simulink model "NREL5MW_FBSWE_SLOW2DOF_AdvancedTorqueController_Part1"  (R2021b)
settings: Solver=ode4  StartTime=0.0  StopTime=Parameter.Time.TMax  FixedStep=Parameter.Time.dt  RelTol=1e-3  EnableMultiTasking=on
values from neighbouring files (symbols this model uses):
  Parameter = NREL5MWDefaultParameter_FBSWE_AvancedTorqueController(Parameter)    [Exercise06_AdvancedTorqueControllerTest.m]    (also in Exercise06_AdvancedTorqueControllerTest_Part1.m = NREL5MWDefaultParameter_FBSWE_AvancedTorqueController_Part1(; Exercise06_SetPointFadingFineTuning.m = NREL5MWDefaultParameter_FBSWE_SetPointFading(Parameter); Exercise06_SetPointFadingFineTuning_Part3.m = NREL5MWDefaultParameter_FBSWE_SetPointFading_Part2(Parameter; Exercise06_SetPointFadingTest.m = NREL5MWDefaultParameter_FBSWE_SetPointFading(Parameter))
libraries: simulink x1
settings Model: Creator=Phoenix_Shao  LastModifiedBy=david
settings SolverCC: AlgebraicLoopSolver=TrustRegion
settings DataIOCC: MaxDataPoints=1000000  SaveFormat=Array  DSMLogging=off  ReturnWorkspaceOutputs=off
settings OptimizationCC: ExpressionDepthLimit=2147483647  InitFltsAndDblsToZero=on  EfficientMapNaN2IntZero=off  LifeSpan=inf
settings DebuggingCC: SaveWithParameterizedLinksMsg=none  UnderspecifiedInitializationDetection=Classic  MergeDetectMultiDrivingBlocksExec=none  SignalResolutionControl=TryResolveAllWithWarning  SolverPrmCheckMsg=warning  MultiTaskDSMMsg=warning  MultiTaskCondExecSysMsg=none  FcnCallInpInsideContextMsg=warning  AllowSymbolicDim=off  StateNameClashWarn=warning  SFUnexpectedBacktrackingDiag=warning  SFNoUnconditionalDefaultTransitionDiag=warning  SFExecutionAtInitializationDiag=none  SFMachineParentedDataDiag=warning  ArithmeticOperatorsInVariantConditions=warning
settings HardwareCC: ProdBitPerPointer=32  ProdBitPerSizeT=32  ProdBitPerPtrDiffT=32  ProdLargestAtomicFloat=None  ProdIntDivRoundTo=Undefined  ProdEndianess=Unspecified  ProdWordSize=32  ProdHWDeviceType=32-bit Generic  TargetBitPerPointer=64  TargetBitPerSizeT=64  TargetBitPerPtrDiffT=64  TargetLongLongMode=on  TargetIntDivRoundTo=Zero  TargetEndianess=LittleEndian  TargetWordSize=64  TargetHWDeviceType=MATLAB Host  ProdEqTarget=off
settings ModelReferenceCC: PropagateSignalLabelsOutOfModel=off
settings SFSimCC: SimUseLocalCustomCode=off  SimParseCustomCode=off  CustomCodeUndefinedFunction=UseInterfaceOnly
settings RTWCC: SystemTargetFile=accel.tlc  TemplateMakefile=accel_default_tmf  RTWVerbose=off  RTWUseLocalCustomCode=off
settings CodeAppCC: MaxIdLength=128  StateflowObjectComments=on
settings STFCustomTargetCC: MATLABClassNameForMDSCustomization=Simulink.SoftwareTarget.TargetSpecificTriggerConfigurationBase  SystemTargetFile=accel.tlc
settings ConfigComp: CovMetricSettings=dw  CovSaveCumulativeToWorkspaceVar=on  CovSaveSingleToWorkspaceVar=on  CovExternalEMLEnable=off

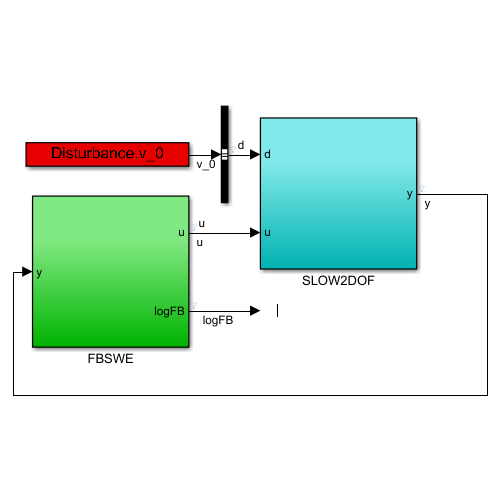
[thumbnail: Simulink's stored preview of the top-level diagram]
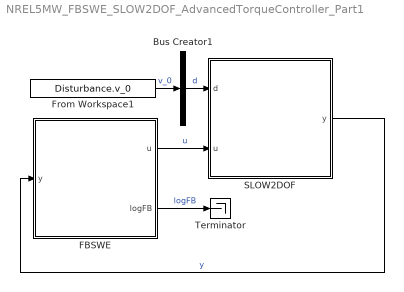
== system NREL5MW_FBSWE_SLOW2DOF_AdvancedTorqueController_Part1 ==
  Bus Creator1 : BusCreator  Inputs=1
  FBSWE : Subsystem
  From Workspace1 : FromWorkspace  VariableName=Disturbance.v_0
  SLOW2DOF : Subsystem
  Terminator : Terminator
  wires:
  FBSWE/1(u) -> SLOW2DOF/2(u)  "u"
  Bus Creator1/1 -> SLOW2DOF/1(d)  "d"
  From Workspace1/1 -> Bus Creator1/1  "v_0"
  SLOW2DOF/1(y) -> FBSWE/1(y)  "y"
  FBSWE/2(logFB) -> Terminator/1  "logFB"

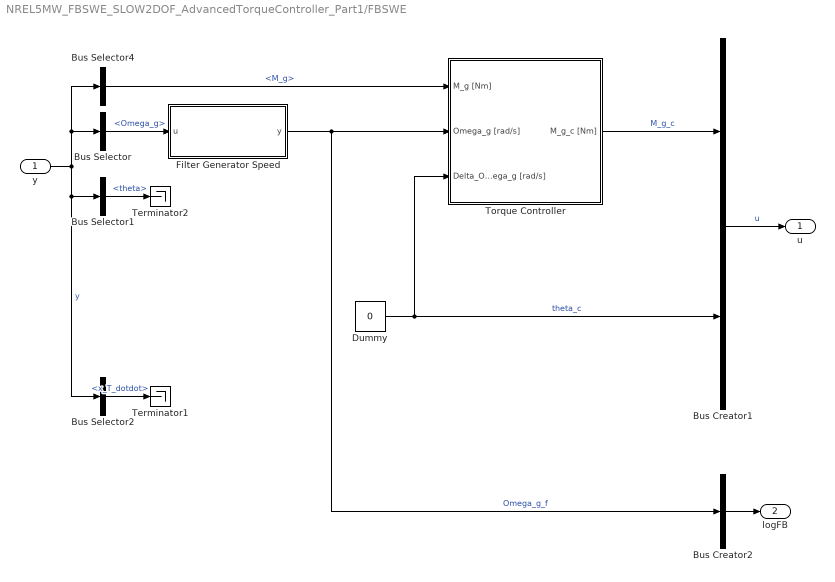
== system NREL5MW_FBSWE_SLOW2DOF_AdvancedTorqueController_Part1/FBSWE ==
  y : Inport
  Bus Creator1 : BusCreator  Inputs=2
  Bus Creator2 : BusCreator  Inputs=1
  Bus Selector : BusSelector  OutputSignals=Omega_g
  Bus Selector1 : BusSelector  OutputSignals=theta
  Bus Selector2 : BusSelector  OutputSignals=x_T_dotdot
  Bus Selector4 : BusSelector  OutputSignals=M_g
  Dummy : Constant  Value=0
  Filter Generator Speed : Subsystem
  Terminator1 : Terminator
  Terminator2 : Terminator
  Torque Controller : Subsystem
  u : Outport  VectorParamsAs1DForOutWhenUnconnected=off
  logFB : Outport  Port=2  VectorParamsAs1DForOutWhenUnconnected=off
  wires:
  Bus Selector/1 -> Filter Generator Speed/1(u)  "<Omega_g>"
  y/1 -> Bus Selector4/1, Bus Selector/1, Bus Selector2/1, Bus Selector1/1  "y"
  Torque Controller/1(M_g_c [Nm]) -> Bus Creator1/1  "M_g_c"
  Bus Creator1/1 -> u/1  "u"
  Filter Generator Speed/1(y) -> Torque Controller/2(Omega_g [rad/s]), Bus Creator2/1  "Omega_g_f"
  Bus Creator2/1 -> logFB/1
  Dummy/1 -> Torque Controller/3(Delta_Omega_g [rad/s]), Bus Creator1/2  "theta_c"
  Bus Selector2/1 -> Terminator1/1  "<x_T_dotdot>"
  Bus Selector1/1 -> Terminator2/1  "<theta>"
  Bus Selector4/1 -> Torque Controller/1(M_g [Nm])  "<M_g>"

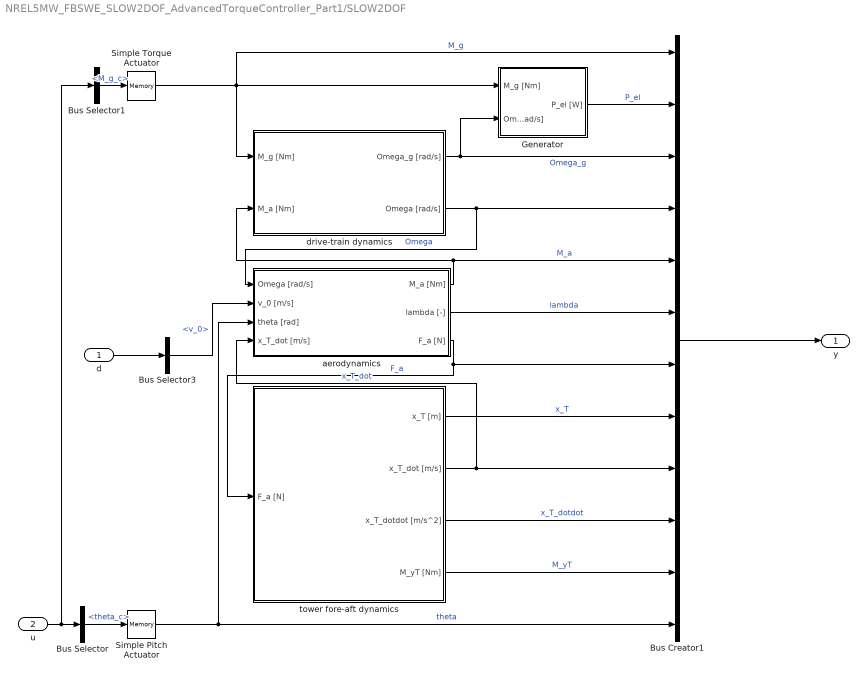
== system NREL5MW_FBSWE_SLOW2DOF_AdvancedTorqueController_Part1/SLOW2DOF ==
  d : Inport
  u : Inport  Port=2
  Bus Creator1 : BusCreator  Inputs=12
  Bus Selector : BusSelector  OutputSignals=theta_c
  Bus Selector1 : BusSelector  OutputSignals=M_g_c
  Bus Selector3 : BusSelector  OutputSignals=v_0
  Generator : Subsystem
  Simple Pitch Actuator : Memory  InitialCondition=Parameter.IC.theta
  Simple Torque Actuator : Memory  InitialCondition=Parameter.IC.M_g
  aerodynamics : Subsystem
  drive-train dynamics : Subsystem
  tower fore-aft dynamics : Subsystem
  y : Outport  VectorParamsAs1DForOutWhenUnconnected=off
  wires:
  Generator/1(P_el [W]) -> Bus Creator1/2  "P_el"
  Bus Creator1/1 -> y/1
  u/1 -> Bus Selector/1, Bus Selector1/1
  Bus Selector/1 -> Simple Pitch Actuator/1  "<theta_c>"
  aerodynamics/3(F_a [N]) -> Bus Creator1/7, tower fore-aft dynamics/1(F_a [N])  "F_a"
  aerodynamics/1(M_a [Nm]) -> Bus Creator1/5, drive-train dynamics/2(M_a [Nm])  "M_a"
  tower fore-aft dynamics/2(x_T_dot [m/s]) -> Bus Creator1/9, aerodynamics/4(x_T_dot [m/s])  "x_T_dot"
  drive-train dynamics/2(Omega [rad/s]) -> Bus Creator1/4, aerodynamics/1(Omega [rad/s])  "Omega"
  drive-train dynamics/1(Omega_g [rad/s]) -> Bus Creator1/3, Generator/2(Omega_g [rad/s])  "Omega_g"
  d/1 -> Bus Selector3/1
  Bus Selector3/1 -> aerodynamics/2(v_0 [m/s])  "<v_0>"
  Simple Pitch Actuator/1 -> Bus Creator1/12, aerodynamics/3(theta [rad])  "theta"
  Bus Selector1/1 -> Simple Torque Actuator/1  "<M_g_c>"
  aerodynamics/2(lambda [-]) -> Bus Creator1/6  "lambda"
  tower fore-aft dynamics/1(x_T [m]) -> Bus Creator1/8  "x_T"
  tower fore-aft dynamics/3(x_T_dotdot [m/s^2]) -> Bus Creator1/10  "x_T_dotdot"
  tower fore-aft dynamics/4(M_yT [Nm]) -> Bus Creator1/11  "M_yT"
  Simple Torque Actuator/1 -> Bus Creator1/1, Generator/1(M_g [Nm]), drive-train dynamics/1(M_g [Nm])  "M_g"

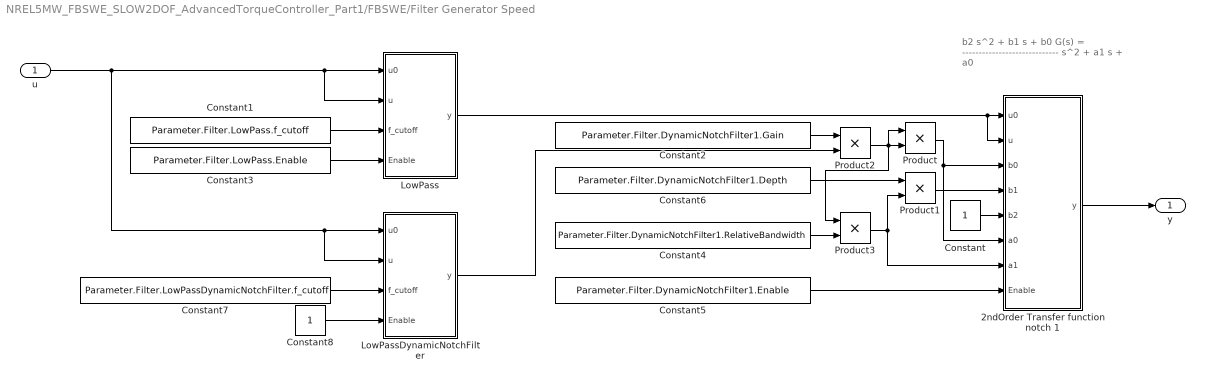
== system NREL5MW_FBSWE_SLOW2DOF_AdvancedTorqueController_Part1/FBSWE/Filter Generator Speed ==
  note: b2 s^2 + b1 s + b0
      | G(s) = -----------------------------
      | s^2 + a1 s + a0
  u : Inport
  2ndOrder Transfer function notch 1 : Subsystem
  Constant : Constant
  Constant1 : Constant  Value=Parameter.Filter.LowPass.f_cutoff
  Constant2 : Constant  Value=Parameter.Filter.DynamicNotchFilter1.Gain
  Constant3 : Constant  Value=Parameter.Filter.LowPass.Enable
  Constant4 : Constant  Value=Parameter.Filter.DynamicNotchFilter1.RelativeBandwidth
  Constant5 : Constant  Value=Parameter.Filter.DynamicNotchFilter1.Enable
  Constant6 : Constant  Value=Parameter.Filter.DynamicNotchFilter1.Depth
  Constant7 : Constant  Value=Parameter.Filter.LowPassDynamicNotchFilter.f_cutoff
  Constant8 : Constant
  LowPass : Subsystem
  LowPassDynamicNotchFilter : Subsystem
  Product{,1..3} (4 alike) : Product  RndMeth=Zero
  y : Outport  VectorParamsAs1DForOutWhenUnconnected=off
  wires:
  Constant3/1 -> LowPass/4(Enable)
  Constant1/1 -> LowPass/3(f_cutoff)
  LowPassDynamicNotchFilter/1(y) -> Product2/2
  Product2/1 -> Product3/1, Product/1, Product/2
  Constant2/1 -> Product2/1
  Constant/1 -> 2ndOrder Transfer function notch 1/5(b2)
  Product1/1 -> 2ndOrder Transfer function notch 1/4(b1)
  2ndOrder Transfer function notch 1/1(y) -> y/1
  Constant4/1 -> Product3/2
  Constant6/1 -> Product1/1
  Product/1 -> 2ndOrder Transfer function notch 1/3(b0), 2ndOrder Transfer function notch 1/6(a0)
  LowPass/1(y) -> 2ndOrder Transfer function notch 1/2(u), 2ndOrder Transfer function notch 1/1(u0)
  Constant5/1 -> 2ndOrder Transfer function notch 1/8(Enable)
  Constant7/1 -> LowPassDynamicNotchFilter/3(f_cutoff)
  Constant8/1 -> LowPassDynamicNotchFilter/4(Enable)
  u/1 -> LowPassDynamicNotchFilter/1(u0), LowPassDynamicNotchFilter/2(u), LowPass/2(u), LowPass/1(u0)
  Product3/1 -> 2ndOrder Transfer function notch 1/7(a1), Product1/2

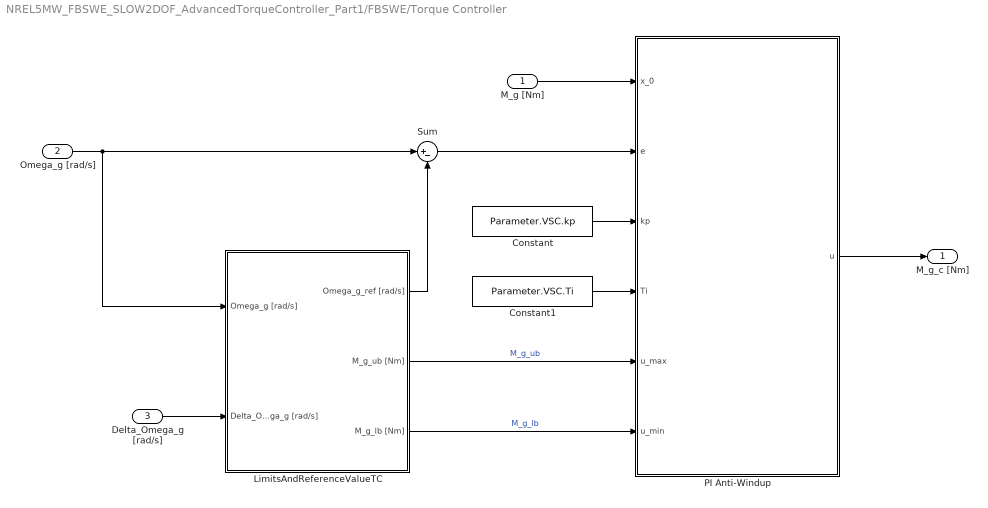
== system NREL5MW_FBSWE_SLOW2DOF_AdvancedTorqueController_Part1/FBSWE/Torque Controller ==
  M_g [Nm] : Inport
  Omega_g [rad/s] : Inport  Port=2
  Delta_Omega_g [rad/s] : Inport  Port=3
  Constant : Constant  Value=Parameter.VSC.kp
  Constant1 : Constant  Value=Parameter.VSC.Ti
  LimitsAndReferenceValueTC : Subsystem
  PI Anti-Windup : Subsystem
  Sum : Sum  Inputs=|+-
  M_g_c [Nm] : Outport  VectorParamsAs1DForOutWhenUnconnected=off
  wires:
  LimitsAndReferenceValueTC/1(Omega_g_ref [rad/s]) -> Sum/2
  M_g [Nm]/1 -> PI Anti-Windup/1(x_0)
  Sum/1 -> PI Anti-Windup/2(e)
  Constant/1 -> PI Anti-Windup/3(kp)
  Constant1/1 -> PI Anti-Windup/4(Ti)
  Omega_g [rad/s]/1 -> LimitsAndReferenceValueTC/1(Omega_g [rad/s]), Sum/1
  LimitsAndReferenceValueTC/2(M_g_ub [Nm]) -> PI Anti-Windup/5(u_max)  "M_g_ub"
  LimitsAndReferenceValueTC/3(M_g_lb [Nm]) -> PI Anti-Windup/6(u_min)  "M_g_lb"
  PI Anti-Windup/1(u) -> M_g_c [Nm]/1
  Delta_Omega_g [rad/s]/1 -> LimitsAndReferenceValueTC/2(Delta_Omega_g [rad/s])

== system NREL5MW_FBSWE_SLOW2DOF_AdvancedTorqueController_Part1/SLOW2DOF/Generator ==
  M_g [Nm] : Inport
  Omega_g [rad/s] : Inport  Port=2
  Constant3 : Constant  Value=Parameter.Generator.eta_el
  Product1 : Product  Inputs=***  RndMeth=Zero
  P_el [W] : Outport  VectorParamsAs1DForOutWhenUnconnected=off
  wires:
  Constant3/1 -> Product1/3
  M_g [Nm]/1 -> Product1/1
  Omega_g [rad/s]/1 -> Product1/2
  Product1/1 -> P_el [W]/1

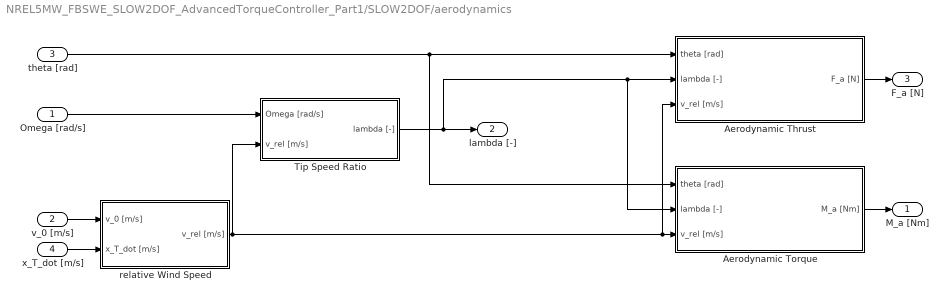
== system NREL5MW_FBSWE_SLOW2DOF_AdvancedTorqueController_Part1/SLOW2DOF/aerodynamics ==
  Omega [rad/s] : Inport
  v_0 [m/s] : Inport  Port=2
  theta [rad] : Inport  Port=3
  x_T_dot [m/s] : Inport  Port=4
  Aerodynamic Thrust : Subsystem
  Aerodynamic Torque : Subsystem
  Tip Speed Ratio : Subsystem
  relative Wind Speed : Subsystem
  M_a [Nm] : Outport  VectorParamsAs1DForOutWhenUnconnected=off
  lambda [-] : Outport  Port=2  VectorParamsAs1DForOutWhenUnconnected=off
  F_a [N] : Outport  Port=3  VectorParamsAs1DForOutWhenUnconnected=off
  wires:
  theta [rad]/1 -> Aerodynamic Thrust/1(theta [rad]), Aerodynamic Torque/1(theta [rad])
  Aerodynamic Torque/1(M_a [Nm]) -> M_a [Nm]/1
  Aerodynamic Thrust/1(F_a [N]) -> F_a [N]/1
  x_T_dot [m/s]/1 -> relative Wind Speed/2(x_T_dot [m/s])
  v_0 [m/s]/1 -> relative Wind Speed/1(v_0 [m/s])
  Omega [rad/s]/1 -> Tip Speed Ratio/1(Omega [rad/s])
  relative Wind Speed/1(v_rel [m/s]) -> Tip Speed Ratio/2(v_rel [m/s]), Aerodynamic Torque/3(v_rel [m/s]), Aerodynamic Thrust/3(v_rel [m/s])
  Tip Speed Ratio/1(lambda [-]) -> Aerodynamic Thrust/2(lambda [-]), Aerodynamic Torque/2(lambda [-]), lambda [-]/1

== system NREL5MW_FBSWE_SLOW2DOF_AdvancedTorqueController_Part1/SLOW2DOF/drive-train dynamics ==
  M_g [Nm] : Inport
  M_a [Nm] : Inport  Port=2
  Add4 : Sum  Inputs=-+
  Gain12 : Gain  Gain=Parameter.Turbine.r_GB  SaturateOnIntegerOverflow=on  OutDataTypeStr=Inherit: Same as input  ParamDataTypeStr=Inherit: Same as input
  Gain2 : Gain  Gain=Parameter.Turbine.r_GB  SaturateOnIntegerOverflow=on  OutDataTypeStr=Inherit: Same as input  ParamDataTypeStr=Inherit: Same as input
  Gain8 : Gain  Gain=1/Parameter.Turbine.J  SaturateOnIntegerOverflow=on  OutDataTypeStr=Inherit: Same as input  ParamDataTypeStr=Inherit: Same as input
  Integrator4 : Integrator  InitialCondition=Parameter.IC.Omega
  Omega_g [rad/s] : Outport  VectorParamsAs1DForOutWhenUnconnected=off
  Omega [rad/s] : Outport  Port=2  VectorParamsAs1DForOutWhenUnconnected=off
  wires:
  M_a [Nm]/1 -> Add4/2  "M_a"
  Integrator4/1 -> Omega [rad/s]/1, Gain12/1  "Omega"
  Add4/1 -> Gain8/1
  Gain8/1 -> Integrator4/1
  Gain2/1 -> Add4/1
  Gain12/1 -> Omega_g [rad/s]/1  "Omega_g [rad/s]"
  M_g [Nm]/1 -> Gain2/1  "M_g"

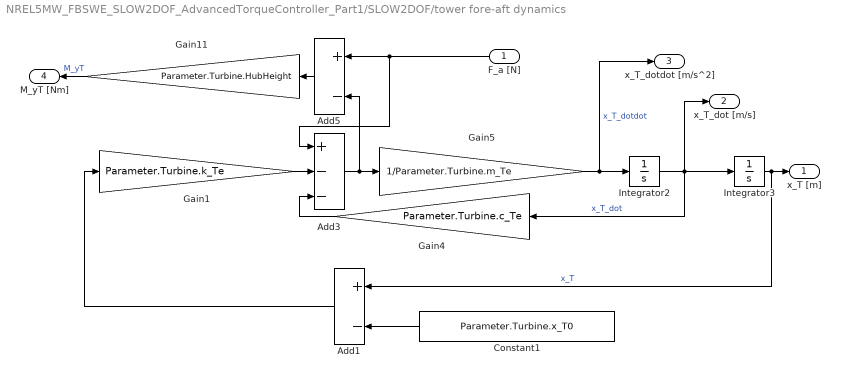
== system NREL5MW_FBSWE_SLOW2DOF_AdvancedTorqueController_Part1/SLOW2DOF/tower fore-aft dynamics ==
  F_a [N] : Inport
  Add1 : Sum  Inputs=+-
  Add3 : Sum  Inputs=+--
  Add5 : Sum  Inputs=+-
  Constant1 : Constant  Value=Parameter.Turbine.x_T0
  Gain1 : Gain  Gain=Parameter.Turbine.k_Te  SaturateOnIntegerOverflow=on  OutDataTypeStr=Inherit: Same as input  ParamDataTypeStr=Inherit: Same as input
  Gain11 : Gain  Gain=Parameter.Turbine.HubHeight  SaturateOnIntegerOverflow=on  OutDataTypeStr=Inherit: Same as input  ParamDataTypeStr=Inherit: Same as input
  Gain4 : Gain  Gain=Parameter.Turbine.c_Te  SaturateOnIntegerOverflow=on  OutDataTypeStr=Inherit: Same as input  ParamDataTypeStr=Inherit: Same as input
  Gain5 : Gain  Gain=1/Parameter.Turbine.m_Te  SaturateOnIntegerOverflow=on  OutDataTypeStr=Inherit: Same as input  ParamDataTypeStr=Inherit: Same as input
  Integrator2 : Integrator
  Integrator3 : Integrator  InitialCondition=Parameter.IC.x_T
  x_T [m] : Outport  VectorParamsAs1DForOutWhenUnconnected=off
  x_T_dot [m/s] : Outport  Port=2  VectorParamsAs1DForOutWhenUnconnected=off
  x_T_dotdot [m/s^2] : Outport  Port=3  VectorParamsAs1DForOutWhenUnconnected=off
  M_yT [Nm] : Outport  Port=4  VectorParamsAs1DForOutWhenUnconnected=off
  wires:
  Constant1/1 -> Add1/2
  Add1/1 -> Gain1/1
  Add3/1 -> Gain5/1, Add5/2
  Integrator2/1 -> Gain4/1, Integrator3/1, x_T_dot [m/s]/1  "x_T_dot"
  Integrator3/1 -> x_T [m]/1, Add1/1  "x_T"
  Gain4/1 -> Add3/3
  Gain1/1 -> Add3/2
  Gain5/1 -> x_T_dotdot [m/s^2]/1, Integrator2/1  "x_T_dotdot"
  Add5/1 -> Gain11/1
  Gain11/1 -> M_yT [Nm]/1  "M_yT"
  F_a [N]/1 -> Add5/1, Add3/1

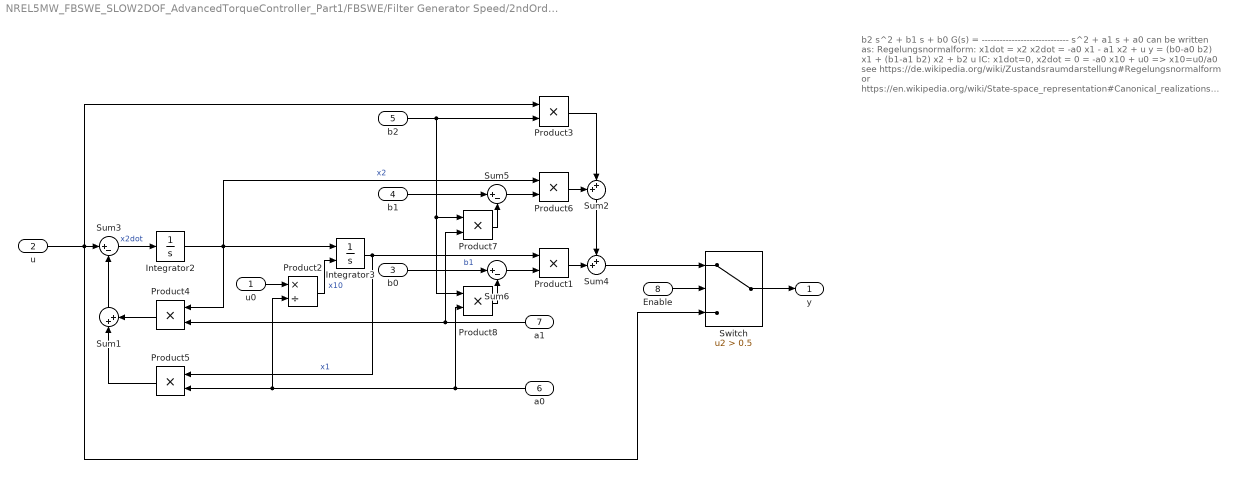
== system NREL5MW_FBSWE_SLOW2DOF_AdvancedTorqueController_Part1/FBSWE/Filter Generator Speed/2ndOrder Transfer function notch 1 ==
  note: b2 s^2 + b1 s + b0
      | G(s) = -----------------------------
      | s^2 + a1 s + a0
      |
      | can be written as:
      |
      | Regelungsnormalform:
      | x1dot = x2
      | x2dot = -a0 x1 - a1 x2 + u
      | y = (b0-a0 b2) x1 + (b1-a1 b2) x2 + b2 u
      |
      | IC: x1dot=0, x2dot = 0 = -a0 x10 + u0 => x10=u0/a0
      |
      | see https://de.wikipedia.org/wiki/Zustandsraumdarstellung#Regelungsnormalform
      | or
      | https://en.wikipedia.org/wiki/State-space_representation#Canonical_realizations
      |
      | Advantage:
      | - IC can be set
      | - coefficients can be changed online
  u0 : Inport
  u : Inport  Port=2
  b0 : Inport  Port=3
  b1 : Inport  Port=4
  b2 : Inport  Port=5
  a0 : Inport  Port=6
  a1 : Inport  Port=7
  Enable : Inport  Port=8
  Integrator2 : Integrator
  Integrator3 : Integrator  InitialConditionSource=external
  Product{1,3..8} (7 alike) : Product  RndMeth=Zero
  Product2 : Product  Inputs=*/  RndMeth=Zero
  Sum1 : Sum  Inputs=|++
  Sum2 : Sum  Inputs=++|
  Sum3 : Sum  Inputs=|+-
  Sum4 : Sum  Inputs=++|
  Sum5 : Sum  Inputs=|+-
  Sum6 : Sum  Inputs=|+-
  Switch : Switch  Criteria=u2 > Threshold  Threshold=0.5
  y : Outport
  wires:
  Switch/1 -> y/1
  Enable/1 -> Switch/2
  Integrator2/1 -> Integrator3/1, Product6/1, Product4/1  "x2"
  Integrator3/1 -> Product1/1, Product5/1  "x1"
  Sum3/1 -> Integrator2/1  "x2dot"
  u/1 -> Product3/1, Sum3/1, Switch/3
  Sum4/1 -> Switch/1
  Product1/1 -> Sum4/2
  Product6/1 -> Sum2/1
  Sum2/1 -> Sum4/1
  Sum1/1 -> Sum3/2
  Product4/1 -> Sum1/2
  Product5/1 -> Sum1/1
  a0/1 -> Product8/2, Product2/2, Product5/2
  a1/1 -> Product7/2, Product4/2
  b2/1 -> Product8/1, Product7/1, Product3/2
  Product3/1 -> Sum2/2
  Sum5/1 -> Product6/2
  b1/1 -> Sum5/1
  Product7/1 -> Sum5/2
  Sum6/1 -> Product1/2
  b0/1 -> Sum6/1  "b1"
  Product8/1 -> Sum6/2
  Product2/1 -> Integrator3/2  "x10"
  u0/1 -> Product2/1

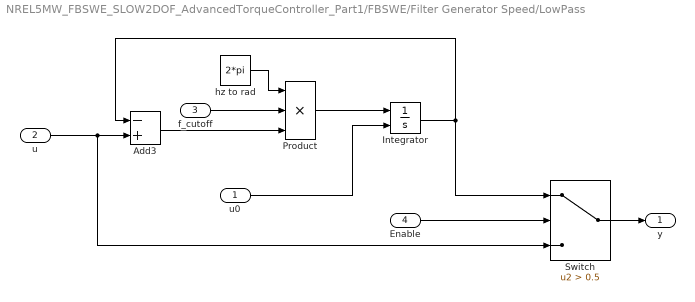
== system NREL5MW_FBSWE_SLOW2DOF_AdvancedTorqueController_Part1/FBSWE/Filter Generator Speed/LowPass ==
  u0 : Inport
  u : Inport  Port=2
  f_cutoff : Inport  Port=3
  Enable : Inport  Port=4
  Add3 : Sum  Inputs=-+
  Integrator : Integrator  InitialConditionSource=external
  Product : Product  Inputs=3  RndMeth=Zero
  Switch : Switch  Criteria=u2 > Threshold  Threshold=0.5
  hz to rad : Constant  Value=2*pi
  y : Outport  VectorParamsAs1DForOutWhenUnconnected=off
  wires:
  u0/1 -> Integrator/2
  Switch/1 -> y/1
  Enable/1 -> Switch/2
  u/1 -> Add3/2, Switch/3
  Integrator/1 -> Switch/1, Add3/1
  Product/1 -> Integrator/1
  Add3/1 -> Product/3
  f_cutoff/1 -> Product/2
  hz to rad/1 -> Product/1

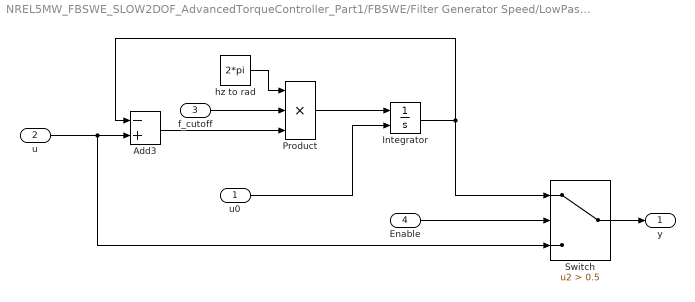
== system NREL5MW_FBSWE_SLOW2DOF_AdvancedTorqueController_Part1/FBSWE/Filter Generator Speed/LowPassDynamicNotchFilter ==
  u0 : Inport
  u : Inport  Port=2
  f_cutoff : Inport  Port=3
  Enable : Inport  Port=4
  Add3 : Sum  Inputs=-+
  Integrator : Integrator  InitialConditionSource=external
  Product : Product  Inputs=3  RndMeth=Zero
  Switch : Switch  Criteria=u2 > Threshold  Threshold=0.5
  hz to rad : Constant  Value=2*pi
  y : Outport  VectorParamsAs1DForOutWhenUnconnected=off
  wires:
  hz to rad/1 -> Product/1
  f_cutoff/1 -> Product/2
  Add3/1 -> Product/3
  Product/1 -> Integrator/1
  Integrator/1 -> Add3/1, Switch/1
  u/1 -> Switch/3, Add3/2
  Enable/1 -> Switch/2
  Switch/1 -> y/1
  u0/1 -> Integrator/2

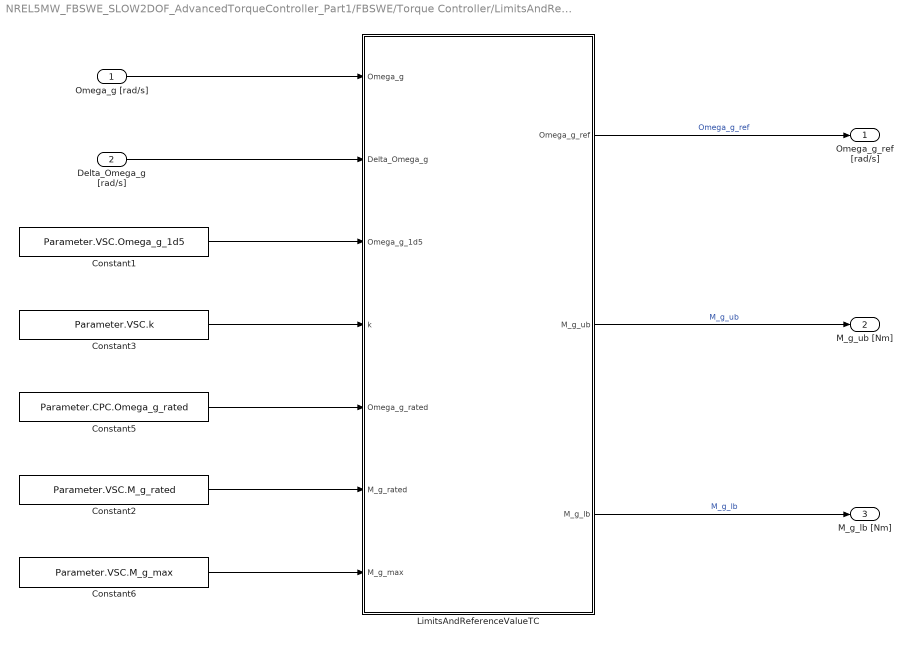
== system NREL5MW_FBSWE_SLOW2DOF_AdvancedTorqueController_Part1/FBSWE/Torque Controller/LimitsAndReferenceValueTC ==
  Omega_g [rad/s] : Inport
  Delta_Omega_g [rad/s] : Inport  Port=2
  Constant1 : Constant  Value=Parameter.VSC.Omega_g_1d5
  Constant2 : Constant  Value=Parameter.VSC.M_g_rated
  Constant3 : Constant  Value=Parameter.VSC.k
  Constant5 : Constant  Value=Parameter.CPC.Omega_g_rated
  Constant6 : Constant  Value=Parameter.VSC.M_g_max
  LimitsAndReferenceValueTC : MATLAB Function  TreatAsAtomicUnit=on
  Omega_g_ref [rad/s] : Outport  VectorParamsAs1DForOutWhenUnconnected=off
  M_g_ub [Nm] : Outport  Port=2  VectorParamsAs1DForOutWhenUnconnected=off
  M_g_lb [Nm] : Outport  Port=3  VectorParamsAs1DForOutWhenUnconnected=off
  wires:
  LimitsAndReferenceValueTC/2(M_g_ub) -> M_g_ub [Nm]/1  "M_g_ub"
  Omega_g [rad/s]/1 -> LimitsAndReferenceValueTC/1(Omega_g)
  Constant1/1 -> LimitsAndReferenceValueTC/3(Omega_g_1d5)
  Constant3/1 -> LimitsAndReferenceValueTC/4(k)
  Constant2/1 -> LimitsAndReferenceValueTC/6(M_g_rated)
  Constant5/1 -> LimitsAndReferenceValueTC/5(Omega_g_rated)
  LimitsAndReferenceValueTC/1(Omega_g_ref) -> Omega_g_ref [rad/s]/1  "Omega_g_ref"
  LimitsAndReferenceValueTC/3(M_g_lb) -> M_g_lb [Nm]/1  "M_g_lb"
  Constant6/1 -> LimitsAndReferenceValueTC/7(M_g_max)
  Delta_Omega_g [rad/s]/1 -> LimitsAndReferenceValueTC/2(Delta_Omega_g)

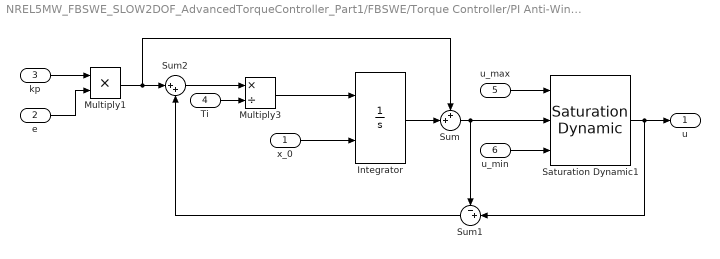
== system NREL5MW_FBSWE_SLOW2DOF_AdvancedTorqueController_Part1/FBSWE/Torque Controller/PI Anti-Windup ==
  x_0 : Inport
  e : Inport  Port=2
  kp : Inport  Port=3
  Ti : Inport  Port=4
  u_max : Inport  Port=5
  u_min : Inport  Port=6
  Integrator : Integrator  InitialConditionSource=external
  Multiply1 : Product  Inputs=**
  Multiply3 : Product  Inputs=*/
  Saturation Dynamic1 : simulink/Discontinuities/Saturation Dynamic  OutMin=[]  OutMax=[]  OutDataTypeStr=Inherit: Same as second input  OutDataType=fixdt(1, 16)  OutScaling=2^-10  DoSatur=off
  Sum : Sum  Inputs=++|
  Sum1 : Sum  Inputs=-+|
  Sum2 : Sum  Inputs=|++
  u : Outport  VectorParamsAs1DForOutWhenUnconnected=off
  wires:
  Saturation Dynamic1/1 -> u/1, Sum1/2
  Integrator/1 -> Sum/2
  kp/1 -> Multiply1/1
  e/1 -> Multiply1/2
  Ti/1 -> Multiply3/2
  Sum1/1 -> Sum2/2
  Multiply1/1 -> Sum/1, Sum2/1
  Sum2/1 -> Multiply3/1
  x_0/1 -> Integrator/2
  Multiply3/1 -> Integrator/1
  u_min/1 -> Saturation Dynamic1/3
  Sum/1 -> Saturation Dynamic1/2, Sum1/1
  u_max/1 -> Saturation Dynamic1/1

== system NREL5MW_FBSWE_SLOW2DOF_AdvancedTorqueController_Part1/SLOW2DOF/aerodynamics/Aerodynamic Thrust ==
  theta [rad] : Inport
  lambda [-] : Inport  Port=2
  v_rel [m/s] : Inport  Port=3
  Fcn1 : Fcn  Expr=1/2*Parameter.General.rho*pi*Parameter.Turbine.R^2*u(1)
  Product1 : Product  Inputs=3  RndMeth=Zero
  effective force coefficient : Lookup2D  RowIndex=Parameter.Turbine.SS.lambda  ColumnIndex=Parameter.Turbine.SS.theta  Table=Parameter.Turbine.SS.c_T
  F_a [N] : Outport  VectorParamsAs1DForOutWhenUnconnected=off
  wires:
  v_rel [m/s]/1 -> Product1/2, Product1/1
  theta [rad]/1 -> effective force coefficient/2
  lambda [-]/1 -> effective force coefficient/1
  Fcn1/1 -> Product1/3
  Product1/1 -> F_a [N]/1  "F_a"
  effective force coefficient/1 -> Fcn1/1  "c_T"

== system NREL5MW_FBSWE_SLOW2DOF_AdvancedTorqueController_Part1/SLOW2DOF/aerodynamics/Aerodynamic Torque ==
  theta [rad] : Inport
  lambda [-] : Inport  Port=2
  v_rel [m/s] : Inport  Port=3
  Fcn1 : Fcn  Expr=1/2*Parameter.General.rho*pi*Parameter.Turbine.R^3*u(1)
  Product1 : Product  Inputs=3  RndMeth=Zero
  Product2 : Product  Inputs=/*  RndMeth=Zero
  effective power coefficient : Lookup2D  RowIndex=Parameter.Turbine.SS.lambda  ColumnIndex=Parameter.Turbine.SS.theta  Table=Parameter.Turbine.SS.c_P
  M_a [Nm] : Outport  VectorParamsAs1DForOutWhenUnconnected=off
  wires:
  Product1/1 -> M_a [Nm]/1  "M_a"
  Fcn1/1 -> Product1/3
  lambda [-]/1 -> effective power coefficient/1, Product2/1
  theta [rad]/1 -> effective power coefficient/2
  v_rel [m/s]/1 -> Product1/1, Product1/2
  effective power coefficient/1 -> Product2/2  "c_P"
  Product2/1 -> Fcn1/1

== system NREL5MW_FBSWE_SLOW2DOF_AdvancedTorqueController_Part1/SLOW2DOF/aerodynamics/Tip Speed Ratio ==
  Omega [rad/s] : Inport
  v_rel [m/s] : Inport  Port=2
  Gain6 : Gain  Gain=Parameter.Turbine.R  SaturateOnIntegerOverflow=on  OutDataTypeStr=Inherit: Same as input  ParamDataTypeStr=Inherit: Same as input
  Product3 : Product  Inputs=*/  RndMeth=Zero
  lambda [-] : Outport  VectorParamsAs1DForOutWhenUnconnected=off
  wires:
  Product3/1 -> Gain6/1
  Omega [rad/s]/1 -> Product3/1
  v_rel [m/s]/1 -> Product3/2
  Gain6/1 -> lambda [-]/1  "lambda"

== system NREL5MW_FBSWE_SLOW2DOF_AdvancedTorqueController_Part1/SLOW2DOF/aerodynamics/relative Wind Speed ==
  v_0 [m/s] : Inport
  x_T_dot [m/s] : Inport  Port=2
  Add2 : Sum  Inputs=-+
  v_rel [m/s] : Outport  VectorParamsAs1DForOutWhenUnconnected=off
  wires:
  Add2/1 -> v_rel [m/s]/1  "v_rel"
  x_T_dot [m/s]/1 -> Add2/1
  v_0 [m/s]/1 -> Add2/2

== matlab function NREL5MW_FBSWE_SLOW2DOF_AdvancedTorqueController_Part1/FBSWE/Torque Controller/LimitsAndReferenceValueTC/LimitsAndReferenceValueTC ==
  settings: fimath=|
      | fimath(...
      | 'RoundMode', 'floor',...
      | 'OverflowMode', 'wrap',...
      | 'ProductMode', 'KeepLSB', 'ProductWordLength', 32,...
      | 'SumMode', 'KeepLSB', 'SumWordLength', 32,...
      | 'CastBeforeSum', false)
  data: Omega_g_ref output; M_g_ub output; M_g_lb output; Omega_g input; Delta_Omega_g input; Omega_g_1d5 input; k input; Omega_g_rated input; M_g_rated input; M_g_max input
function [Omega_g_ref,M_g_ub,M_g_lb] = LimitsAndReferenceValueTC(...
    Omega_g,Delta_Omega_g,...               % signals
    Omega_g_1d5,...                         % Region 1.5 parameters
    k,...                                   % Region   2 parameters
    Omega_g_rated,...                       % Region 2.5 parameters
    M_g_rated,...                           % Region   3 parameters
    M_g_max)                                % limits
 


%% Internals
Omega_g_R2Switch    = 0.5*(Omega_g_1d5 + Omega_g_rated);   % switch speed between Region 1.5 and 2.5

%% State Machine
if Omega_g < Omega_g_R2Switch
    % Region 1.5: speed reference is the minimum speed
    % torque limits: 0 ... optimal torque (Region 2 curve)
    Omega_g_ref = Omega_g_1d5;
    M_g_lb      = 0;
    M_g_ub      = k*Omega_g^2;
else
    % Region 2.5: speed reference is rated generator speed
    % torque limits: optimal torque ... rated torque (constant power), capped at M_g_max
    Omega_g_ref = Omega_g_rated;
    M_g_lb      = k*Omega_g^2;
    M_g_ub      = min(M_g_rated*Omega_g_rated/max(Omega_g,1e-6), M_g_max);
end

end
